simulink library "lpvcoreLibraryCore"  (R2020a)
settings: Solver=VariableStepAuto  StartTime=0.0  StopTime=10.0  RelTol=1e-3
undefined symbols (not defined in the file or in its folder): __PRM__SERIALIZED__DATA__, lpvlfr, lpvss, M, P, pmatrix
libraries: $bdroot x2
settings Model: Creator=Patrick  LastModifiedBy=Patrick

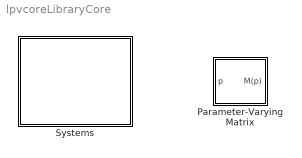
== system lpvcoreLibraryCore ==
  Parameter-Varying Matrix : Subsystem  BlockKeywords=__PRM__SERIALIZED__DATA__:pmatrix  mask(Parameter-Varying Matrix){M=M}
      mask prompts: M "Parameter-varying matrix (pmatrix):"
      mask help: Evaluates parameter-varying matrix according to the input.
      mask init:
      | [nm,nn] = size(M);
      | np = M.Np;
      | 
      | % 'Fix' in case empty pmatrix object is given
      | if nm*nn == 0
      |     % Create constant scalar pmatrix object
      |     M = 0*preal('p');
      |     np = 1;
      |     nm = 1;
      |     nn = 1;
      | end
      mask Help:
      | The Parameter-Varying Matrix block evaluates a pmatrix object (see 'help pmatrix') according to the input given to the block.
      | 
      | Block input:
      | 	p (double): The value of the scheduling-variable the parameter-varying matrix should be evaluated at.
      | 
      | Block output:
      | 	M (double): Value of the parameter-varying matrix for the value of the scheduling-variable p.
      mask DialogControl DescGroupVar Prompt: Parameter-Varying Matrix
      mask DialogControl DescTextVar Prompt: Evaluates parameter-varying matrix according to the input.
      mask Display:
      | port_label('input',1,'p')
      | port_label('output',1,'M(p)')
  Systems : Subsystem  Description=Test  mask(System blocks){}

== system lpvcoreLibraryCore/Parameter-Varying Matrix ==
  p : Inport
  Reshape : Reshape  OutputDimensionality=Customize  OutputDimensions=[nm,nn]
  S-Function : S-Function  FunctionName=sfunEvalMat  Parameters=M,nm,nn,np  SFunctionDeploymentMode=off  EnableBusSupport=off
  M(p) : Outport
  wires:
  Reshape/1 -> M(p)/1
  S-Function/1 -> Reshape/1
  p/1 -> S-Function/1

== system lpvcoreLibraryCore/Systems ==
  Continuous Time LPV System : Subsystem  BlockKeywords=__PRM__SERIALIZED__DATA__:lpvss,lpvlfr  mask(Continuous Time LPV System){P=P, x0=0, stateOut=off}
      mask prompts: P "System:"; stateOut "State output"
      mask help: Simulates continuous time LPV system.
      mask init:
      | %% Add state-output if option is active
      | block = find_system(gcb,...
      |           'LookUnderMasks','on',...
      |           'FollowLinks','on','Name','xout');
      | blockTerminator = find_system(gcb,...
      |           'LookUnderMasks','on',...
      |           'FollowLinks','on','Name','Terminator');
      | 
      | if ~stateOut
      |     if ~isempty(block)
      |         delete_block(block);
      |     end
      |     if isempty(blockTerminator)
      |         add_block('built-in/Terminator',[gcb,'/Terminator']);
      |     end
      | else
      |     if ~isempty(blockTerminator)
      |         delete_block(blockTerminator)
      |     end
      |     if isempty(block)
      |         add_block('built-in/Outport',[gcb,'/xout']);
      |     end
      | end
      | 
      | % 'Fix' in case system is LTI, as simulink does not support empty signals
      | if P.Np == 0
      |     % Create system with non-empty Delta block 
      |     P = lpvlfr(0*preal('p'),blkdiag(0,P.G));
      | end
      mask Help:
      | The Continuous Time LPV System block simulates a LPV system represented by a lpvss or lpvlfr object (see 'help lpvss' and 'help lpvlfr') for the input u and the scheduling parameter p.
      | 
      | Block inputs:
      | 	u (double): The input to the LPV system.
      | 	p (double): The scheduling parameter of the LPV system.
      | 
      | Block outputs:
      | 	y (double): Output of the LPV system.
      mask DialogControl DescriptionGroup Prompt: LPV System
      mask DialogControl Control1 Prompt: Simulates continuous time LPV system  described as <a href="matlab:doc lpvss">lpvss</a> or <a href="matlab:doc lpvlfr">lpvlfr</a> object.
      mask DialogControl OptionGroup Prompt: Options
      mask Display:
      | fprintf('LPV System')
      | port_label('input',1,'u')
      | port_label('input',2,'p')
      | port_label('output',1,'y')
      | if stateOut
      |     port_label('output',2,'x')
      | end
  Discrete Time LPV System : Subsystem  BlockKeywords=__PRM__SERIALIZED__DATA__:lpvss,lpvlfr  mask(Discrete Time LPV System){P=P, x0=0, stateOut=off}
      mask prompts: P "System:"; stateOut "State output"
      mask help: Simulates discrete time LPV system.
      mask init:
      | %% Add state-output if option is active
      | block = find_system(gcb,...
      |           'LookUnderMasks','on',...
      |           'FollowLinks','on','Name','xout');
      | blockTerminator = find_system(gcb,...
      |           'LookUnderMasks','on',...
      |           'FollowLinks','on','Name','Terminator');
      | 
      | if ~stateOut
      |     if ~isempty(block)
      |         delete_block(block);
      |     end
      |     if isempty(blockTerminator)
      |         add_block('built-in/Terminator',[gcb,'/Terminator']);
      |     end
      | else
      |     if ~isempty(blockTerminator)
      |         delete_block(blockTerminator)
      |     end
      |     if isempty(block)
      |         add_block('built-in/Outport',[gcb,'/xout']);
      |     end
      | end
      | 
      | % 'Fix' in case system is LTI, as simulink does not support empty signals
      | if P.Np == 0
      |     % Create system with non-empty Delta block 
      |     P = lpvlfr(0*preal('p','dt'),blkdiag(0,P.G));
      | end
      mask Help:
      | The Discrete Time LPV System block simulates a LPV system represented by a lpvss or lpvlfr object (see 'help lpvss' and 'help lpvlfr') for the input u and the scheduling parameter p.
      | 
      | Block inputs:
      | 	u (double): The input to the LPV system.
      | 	p (double): The scheduling parameter of the LPV system.
      | 
      | Block outputs:
      | 	y (double): Output of the LPV system.
      mask DialogControl DescriptionGroup Prompt: LPV System
      mask DialogControl Control1 Prompt: Simulates discrete time LPV system  described as <a href="matlab:doc lpvss">lpvss</a> or <a href="matlab:doc lpvlfr">lpvlfr</a> object.
      mask DialogControl OptionGroup Prompt: Options
      mask Display:
      | fprintf('LPV System')
      | port_label('input',1,'u')
      | port_label('input',2,'p')
      | port_label('output',1,'y')
      | if stateOut
      |     port_label('output',2,'x')
      | end

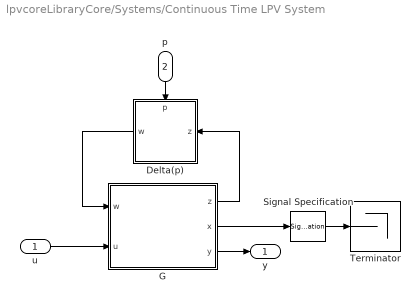
== system lpvcoreLibraryCore/Systems/Continuous Time LPV System ==
  u : Inport
  p : Inport  Port=2
  Delta(p) : Subsystem
      settings: PortSchema="{\"entries\":[{\"content\":{\"sides\":[{\"content\":{\"connectorIds\":[\"In1\"]},\"type\":\"ConnectorPlacement.EquallySpacedRectSide\",\"uuid\":\"40b17919-8477-4d5a-bc1e-07124560e0a8\"},{\"content\":{\"connectorIds\":[\"Out1\"],\"side\":\"RIGHT\"},\"type\":\"ConnectorPlacement.EquallySpacedRectSide\",\"uuid\":\"7a9266a5-a008-4440-9d20-97e11119cc78\"},{\"content\":{\"connectorIds\":[],\"side\":\"TOP\"},\"type\":\"ConnectorPlacement.EquallySpacedRectSide\",\"uuid\":\"31a76025-289d-4dd3-b5a5-f1250f01b9a0\"},{\"content\":{\"connectorIds\":[\"In2\"],\"side\":\"BOTTOM\"},\"type\":\"ConnectorPlacement.EquallySpacedRectSide\",\"uuid\":\"e94679d6-bb1b-4760-a84e-ace825484444\"}]},\"type\":\"ConnectorPlacement.EquallySpacedConnector\",\"uuid\":\"6d9e1dd3-84ed-4af3-8c83-c495de9c3e59\"}],\"packageUris\":[\"http://schema.mathworks.com/mf0/Connector/19700101\"],\"version\":\"1.0\"}"
  G : Subsystem
  Signal Specification : SignalSpecification  Dimensions=P.Nx
  Terminator : Terminator
  y : Outport  PortDimensions=P.Ny
  wires:
  G/2(x) -> Signal Specification/1
  G/3(y) -> y/1
  p/1 -> Delta(p)/2(p)
  Signal Specification/1 -> Terminator/1
  G/1(z) -> Delta(p)/1(z)
  Delta(p)/1(w) -> G/1(w)
  u/1 -> G/2(u)

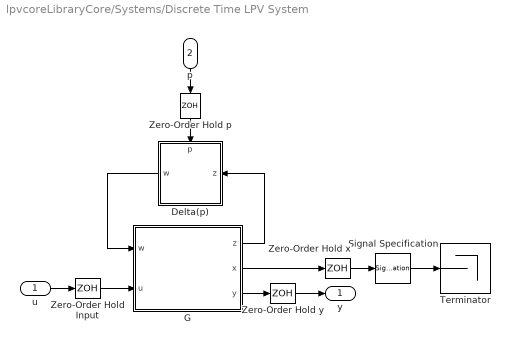
== system lpvcoreLibraryCore/Systems/Discrete Time LPV System ==
  u : Inport
  p : Inport  Port=2
  Delta(p) : Subsystem
      settings: PortSchema="{\"entries\":[{\"content\":{\"sides\":[{\"content\":{\"connectorIds\":[\"In1\"]},\"type\":\"ConnectorPlacement.EquallySpacedRectSide\",\"uuid\":\"40b17919-8477-4d5a-bc1e-07124560e0a8\"},{\"content\":{\"connectorIds\":[\"Out1\"],\"side\":\"RIGHT\"},\"type\":\"ConnectorPlacement.EquallySpacedRectSide\",\"uuid\":\"7a9266a5-a008-4440-9d20-97e11119cc78\"},{\"content\":{\"connectorIds\":[],\"side\":\"TOP\"},\"type\":\"ConnectorPlacement.EquallySpacedRectSide\",\"uuid\":\"31a76025-289d-4dd3-b5a5-f1250f01b9a0\"},{\"content\":{\"connectorIds\":[\"In2\"],\"side\":\"BOTTOM\"},\"type\":\"ConnectorPlacement.EquallySpacedRectSide\",\"uuid\":\"e94679d6-bb1b-4760-a84e-ace825484444\"}]},\"type\":\"ConnectorPlacement.EquallySpacedConnector\",\"uuid\":\"6d9e1dd3-84ed-4af3-8c83-c495de9c3e59\"}],\"packageUris\":[\"http://schema.mathworks.com/mf0/Connector/19700101\"],\"version\":\"1.0\"}"
  G : Subsystem
  Signal Specification : SignalSpecification  Dimensions=P.Nx  SampleTime=P.Ts
  Terminator : Terminator
  Zero-Order Hold Input : ZeroOrderHold  SampleTime=P.Ts
  Zero-Order Hold p : ZeroOrderHold  SampleTime=P.Ts
  Zero-Order Hold x : ZeroOrderHold  SampleTime=P.Ts
  Zero-Order Hold y : ZeroOrderHold  SampleTime=P.Ts
  y : Outport  PortDimensions=P.Ny  SampleTime=P.Ts
  wires:
  G/2(x) -> Zero-Order Hold x/1
  G/3(y) -> Zero-Order Hold y/1
  u/1 -> Zero-Order Hold Input/1
  p/1 -> Zero-Order Hold p/1
  Signal Specification/1 -> Terminator/1
  Zero-Order Hold y/1 -> y/1
  Zero-Order Hold x/1 -> Signal Specification/1
  Delta(p)/1(w) -> G/1(w)
  Zero-Order Hold Input/1 -> G/2(u)
  G/1(z) -> Delta(p)/1(z)
  Zero-Order Hold p/1 -> Delta(p)/2(p)

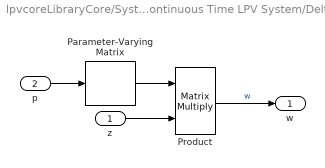
== system lpvcoreLibraryCore/Systems/Continuous Time LPV System/Delta(p) ==
  z : Inport
  p : Inport  Port=2
  Parameter-Varying Matrix : $bdroot/Parameter-Varying Matrix  M=P.Delta
  Product : Product  Multiplication=Matrix(*)
  w : Outport
  wires:
  Product/1 -> w/1  "w"
  z/1 -> Product/2
  p/1 -> Parameter-Varying Matrix/1
  Parameter-Varying Matrix/1 -> Product/1

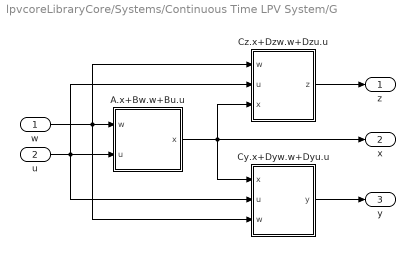
== system lpvcoreLibraryCore/Systems/Continuous Time LPV System/G ==
  w : Inport
  u : Inport  Port=2
  A.x+Bw.w+Bu.u : Subsystem
  Cy.x+Dyw.w+Dyu.u : Subsystem
      settings: PortSchema="{\"entries\":[{\"content\":{\"sides\":[{\"content\":{\"connectorIds\":[]},\"type\":\"ConnectorPlacement.EquallySpacedRectSide\",\"uuid\":\"cff2ddf5-991f-421a-8c0b-791ed633647a\"},{\"content\":{\"connectorIds\":[],\"side\":\"RIGHT\"},\"type\":\"ConnectorPlacement.EquallySpacedRectSide\",\"uuid\":\"64d1d737-6a99-44bb-a50e-22ad775baef2\"},{\"content\":{\"connectorIds\":[\"In1\",\"In2\",\"In3\"],\"side\":\"TOP\"},\"type\":\"ConnectorPlacement.EquallySpacedRectSide\",\"uuid\":\"55fd9704-b08d-4aec-b8d4-8557118b3529\"},{\"content\":{\"connectorIds\":[\"Out1\"],\"side\":\"BOTTOM\"},\"type\":\"ConnectorPlacement.EquallySpacedRectSide\",\"uuid\":\"9cdd13fd-e3e4-4b56-b008-ec31afd91319\"}]},\"type\":\"ConnectorPlacement.EquallySpacedConnector\",\"uuid\":\"58a3a2c5-2630-4247-8a21-26ad04b014a8\"}],\"packageUris\":[\"http://schema.mathworks.com/mf0/Connector/19700101\"],\"version\":\"1.0\"}"
  Cz.x+Dzw.w+Dzu.u : Subsystem
      settings: PortSchema="{\"entries\":[{\"content\":{\"sides\":[{\"content\":{\"connectorIds\":[]},\"type\":\"ConnectorPlacement.EquallySpacedRectSide\",\"uuid\":\"cff2ddf5-991f-421a-8c0b-791ed633647a\"},{\"content\":{\"connectorIds\":[],\"side\":\"RIGHT\"},\"type\":\"ConnectorPlacement.EquallySpacedRectSide\",\"uuid\":\"64d1d737-6a99-44bb-a50e-22ad775baef2\"},{\"content\":{\"connectorIds\":[\"In1\",\"In2\",\"In3\"],\"side\":\"TOP\"},\"type\":\"ConnectorPlacement.EquallySpacedRectSide\",\"uuid\":\"55fd9704-b08d-4aec-b8d4-8557118b3529\"},{\"content\":{\"connectorIds\":[\"Out1\"],\"side\":\"BOTTOM\"},\"type\":\"ConnectorPlacement.EquallySpacedRectSide\",\"uuid\":\"c5f26be2-8a20-4d52-a73e-a9231d806b06\"}]},\"type\":\"ConnectorPlacement.EquallySpacedConnector\",\"uuid\":\"58a3a2c5-2630-4247-8a21-26ad04b014a8\"}],\"packageUris\":[\"http://schema.mathworks.com/mf0/Connector/19700101\"],\"version\":\"1.0\"}"
  z : Outport
  x : Outport  Port=2
  y : Outport  Port=3
  wires:
  Cy.x+Dyw.w+Dyu.u/1(y) -> y/1
  A.x+Bw.w+Bu.u/1(x) -> Cy.x+Dyw.w+Dyu.u/3(x), Cz.x+Dzw.w+Dzu.u/1(x), x/1
  Cz.x+Dzw.w+Dzu.u/1(z) -> z/1
  u/1 -> Cz.x+Dzw.w+Dzu.u/2(u), Cy.x+Dyw.w+Dyu.u/2(u), A.x+Bw.w+Bu.u/2(u)
  w/1 -> Cy.x+Dyw.w+Dyu.u/1(w), Cz.x+Dzw.w+Dzu.u/3(w), A.x+Bw.w+Bu.u/1(w)

== system lpvcoreLibraryCore/Systems/Discrete Time LPV System/Delta(p) ==
  z : Inport
  p : Inport  Port=2
  Parameter-Varying Matrix : $bdroot/Parameter-Varying Matrix  M=P.Delta
  Product : Product  Multiplication=Matrix(*)
  w : Outport
  wires:
  Product/1 -> w/1  "w"
  z/1 -> Product/2
  p/1 -> Parameter-Varying Matrix/1
  Parameter-Varying Matrix/1 -> Product/1

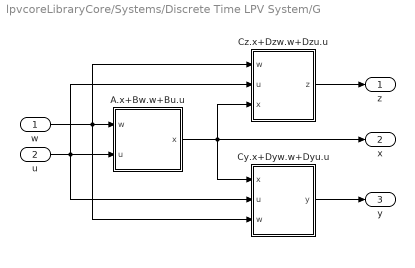
== system lpvcoreLibraryCore/Systems/Discrete Time LPV System/G ==
  w : Inport
  u : Inport  Port=2
  A.x+Bw.w+Bu.u : Subsystem
  Cy.x+Dyw.w+Dyu.u : Subsystem
      settings: PortSchema="{\"entries\":[{\"content\":{\"sides\":[{\"content\":{\"connectorIds\":[]},\"type\":\"ConnectorPlacement.EquallySpacedRectSide\",\"uuid\":\"cff2ddf5-991f-421a-8c0b-791ed633647a\"},{\"content\":{\"connectorIds\":[],\"side\":\"RIGHT\"},\"type\":\"ConnectorPlacement.EquallySpacedRectSide\",\"uuid\":\"64d1d737-6a99-44bb-a50e-22ad775baef2\"},{\"content\":{\"connectorIds\":[\"In1\",\"In2\",\"In3\"],\"side\":\"TOP\"},\"type\":\"ConnectorPlacement.EquallySpacedRectSide\",\"uuid\":\"55fd9704-b08d-4aec-b8d4-8557118b3529\"},{\"content\":{\"connectorIds\":[\"Out1\"],\"side\":\"BOTTOM\"},\"type\":\"ConnectorPlacement.EquallySpacedRectSide\",\"uuid\":\"9cdd13fd-e3e4-4b56-b008-ec31afd91319\"}]},\"type\":\"ConnectorPlacement.EquallySpacedConnector\",\"uuid\":\"58a3a2c5-2630-4247-8a21-26ad04b014a8\"}],\"packageUris\":[\"http://schema.mathworks.com/mf0/Connector/19700101\"],\"version\":\"1.0\"}"
  Cz.x+Dzw.w+Dzu.u : Subsystem
      settings: PortSchema="{\"entries\":[{\"content\":{\"sides\":[{\"content\":{\"connectorIds\":[]},\"type\":\"ConnectorPlacement.EquallySpacedRectSide\",\"uuid\":\"cff2ddf5-991f-421a-8c0b-791ed633647a\"},{\"content\":{\"connectorIds\":[],\"side\":\"RIGHT\"},\"type\":\"ConnectorPlacement.EquallySpacedRectSide\",\"uuid\":\"64d1d737-6a99-44bb-a50e-22ad775baef2\"},{\"content\":{\"connectorIds\":[\"In1\",\"In2\",\"In3\"],\"side\":\"TOP\"},\"type\":\"ConnectorPlacement.EquallySpacedRectSide\",\"uuid\":\"55fd9704-b08d-4aec-b8d4-8557118b3529\"},{\"content\":{\"connectorIds\":[\"Out1\"],\"side\":\"BOTTOM\"},\"type\":\"ConnectorPlacement.EquallySpacedRectSide\",\"uuid\":\"c5f26be2-8a20-4d52-a73e-a9231d806b06\"}]},\"type\":\"ConnectorPlacement.EquallySpacedConnector\",\"uuid\":\"58a3a2c5-2630-4247-8a21-26ad04b014a8\"}],\"packageUris\":[\"http://schema.mathworks.com/mf0/Connector/19700101\"],\"version\":\"1.0\"}"
  z : Outport
  x : Outport  Port=2
  y : Outport  Port=3
  wires:
  Cy.x+Dyw.w+Dyu.u/1(y) -> y/1
  A.x+Bw.w+Bu.u/1(x) -> Cy.x+Dyw.w+Dyu.u/3(x), Cz.x+Dzw.w+Dzu.u/1(x), x/1
  Cz.x+Dzw.w+Dzu.u/1(z) -> z/1
  u/1 -> Cz.x+Dzw.w+Dzu.u/2(u), Cy.x+Dyw.w+Dyu.u/2(u), A.x+Bw.w+Bu.u/2(u)
  w/1 -> Cy.x+Dyw.w+Dyu.u/1(w), Cz.x+Dzw.w+Dzu.u/3(w), A.x+Bw.w+Bu.u/1(w)

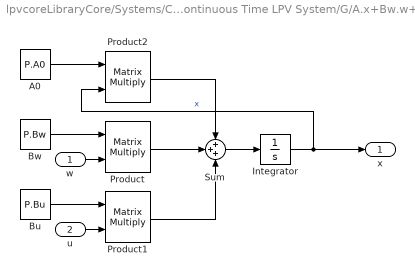
== system lpvcoreLibraryCore/Systems/Continuous Time LPV System/G/A.x+Bw.w+Bu.u ==
  w : Inport
  u : Inport  Port=2
  A0 : Constant  Value=P.A0  VectorParams1D=off
  Bu : Constant  Value=P.Bu  VectorParams1D=off
  Bw : Constant  Value=P.Bw  VectorParams1D=off
  Integrator : Integrator  InitialCondition=x0
  Product : Product  Multiplication=Matrix(*)
  Product1 : Product  Multiplication=Matrix(*)
  Product2 : Product  Multiplication=Matrix(*)
  Sum : Sum  Inputs=+++
  x : Outport
  wires:
  u/1 -> Product1/2
  Product1/1 -> Sum/3
  Integrator/1 -> x/1, Product2/2  "x"
  Product2/1 -> Sum/1
  w/1 -> Product/2
  Bw/1 -> Product/1
  Sum/1 -> Integrator/1
  A0/1 -> Product2/1
  Bu/1 -> Product1/1
  Product/1 -> Sum/2

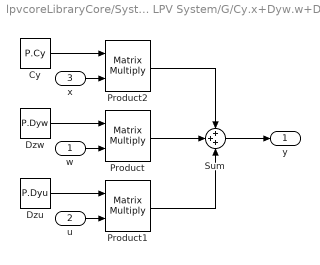
== system lpvcoreLibraryCore/Systems/Continuous Time LPV System/G/Cy.x+Dyw.w+Dyu.u ==
  w : Inport
  u : Inport  Port=2
  x : Inport  Port=3
  Cy : Constant  Value=P.Cy  VectorParams1D=off
  Dzu : Constant  Value=P.Dyu  VectorParams1D=off
  Dzw : Constant  Value=P.Dyw  VectorParams1D=off
  Product : Product  Multiplication=Matrix(*)
  Product1 : Product  Multiplication=Matrix(*)
  Product2 : Product  Multiplication=Matrix(*)
  Sum : Sum  Inputs=+++
  y : Outport
  wires:
  u/1 -> Product1/2
  Product1/1 -> Sum/3
  Product2/1 -> Sum/1
  w/1 -> Product/2
  Dzw/1 -> Product/1
  Cy/1 -> Product2/1
  Dzu/1 -> Product1/1
  Product/1 -> Sum/2
  x/1 -> Product2/2
  Sum/1 -> y/1

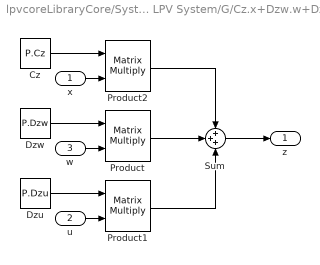
== system lpvcoreLibraryCore/Systems/Continuous Time LPV System/G/Cz.x+Dzw.w+Dzu.u ==
  x : Inport
  u : Inport  Port=2
  w : Inport  Port=3
  Cz : Constant  Value=P.Cz  VectorParams1D=off
  Dzu : Constant  Value=P.Dzu  VectorParams1D=off
  Dzw : Constant  Value=P.Dzw  VectorParams1D=off
  Product : Product  Multiplication=Matrix(*)
  Product1 : Product  Multiplication=Matrix(*)
  Product2 : Product  Multiplication=Matrix(*)
  Sum : Sum  Inputs=+++
  z : Outport
  wires:
  u/1 -> Product1/2
  Product1/1 -> Sum/3
  Product2/1 -> Sum/1
  w/1 -> Product/2
  Dzw/1 -> Product/1
  Cz/1 -> Product2/1
  Dzu/1 -> Product1/1
  Product/1 -> Sum/2
  x/1 -> Product2/2
  Sum/1 -> z/1

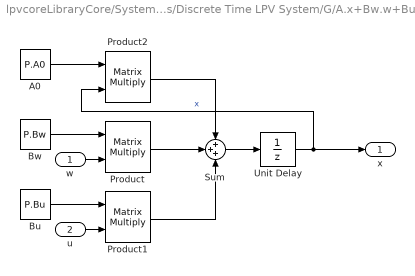
== system lpvcoreLibraryCore/Systems/Discrete Time LPV System/G/A.x+Bw.w+Bu.u ==
  w : Inport
  u : Inport  Port=2
  A0 : Constant  Value=P.A0  VectorParams1D=off
  Bu : Constant  Value=P.Bu  VectorParams1D=off
  Bw : Constant  Value=P.Bw  VectorParams1D=off
  Product : Product  Multiplication=Matrix(*)
  Product1 : Product  Multiplication=Matrix(*)
  Product2 : Product  Multiplication=Matrix(*)
  Sum : Sum  Inputs=+++
  Unit Delay : UnitDelay  InitialCondition=x0  SampleTime=-1  HasFrameUpgradeWarning=on
  x : Outport
  wires:
  u/1 -> Product1/2
  Product1/1 -> Sum/3
  Unit Delay/1 -> x/1, Product2/2  "x"
  Product2/1 -> Sum/1
  w/1 -> Product/2
  Bw/1 -> Product/1
  Sum/1 -> Unit Delay/1
  A0/1 -> Product2/1
  Bu/1 -> Product1/1
  Product/1 -> Sum/2

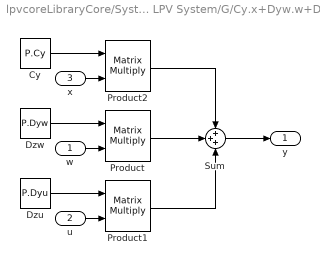
== system lpvcoreLibraryCore/Systems/Discrete Time LPV System/G/Cy.x+Dyw.w+Dyu.u ==
  w : Inport
  u : Inport  Port=2
  x : Inport  Port=3
  Cy : Constant  Value=P.Cy  VectorParams1D=off
  Dzu : Constant  Value=P.Dyu  VectorParams1D=off
  Dzw : Constant  Value=P.Dyw  VectorParams1D=off
  Product : Product  Multiplication=Matrix(*)
  Product1 : Product  Multiplication=Matrix(*)
  Product2 : Product  Multiplication=Matrix(*)
  Sum : Sum  Inputs=+++
  y : Outport
  wires:
  u/1 -> Product1/2
  Product1/1 -> Sum/3
  Product2/1 -> Sum/1
  w/1 -> Product/2
  Dzw/1 -> Product/1
  Cy/1 -> Product2/1
  Dzu/1 -> Product1/1
  Product/1 -> Sum/2
  x/1 -> Product2/2
  Sum/1 -> y/1

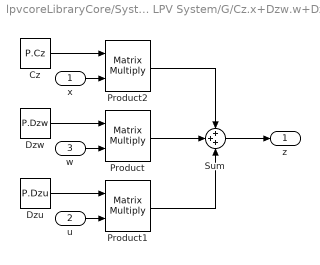
== system lpvcoreLibraryCore/Systems/Discrete Time LPV System/G/Cz.x+Dzw.w+Dzu.u ==
  x : Inport
  u : Inport  Port=2
  w : Inport  Port=3
  Cz : Constant  Value=P.Cz  VectorParams1D=off
  Dzu : Constant  Value=P.Dzu  VectorParams1D=off
  Dzw : Constant  Value=P.Dzw  VectorParams1D=off
  Product : Product  Multiplication=Matrix(*)
  Product1 : Product  Multiplication=Matrix(*)
  Product2 : Product  Multiplication=Matrix(*)
  Sum : Sum  Inputs=+++
  z : Outport
  wires:
  u/1 -> Product1/2
  Product1/1 -> Sum/3
  Product2/1 -> Sum/1
  w/1 -> Product/2
  Dzw/1 -> Product/1
  Cz/1 -> Product2/1
  Dzu/1 -> Product1/1
  Product/1 -> Sum/2
  x/1 -> Product2/2
  Sum/1 -> z/1
